simulink model "LEDblink_v02"  (Simulink 7.1)
settings: Solver=FixedStepDiscrete  StartTime=0.0  StopTime=10.0  FixedStep=0.001  RelTol=1e-3
libraries: dsPICdrivers x4, simulink x1
settings Model: Creator=Lubin  LastModifiedBy=Lubin
settings OptimizationCC: OptimizeModelRefInitCode=on  LifeSpan=1
settings DebuggingCC: SaveWithParameterizedLinksMsg=none  SignalResolutionControl=TryResolveAllWithWarning  MultiTaskDSMMsg=warning  MultiTaskCondExecSysMsg=none
settings HardwareCC: ProdBitPerInt=16  ProdEndianess=LittleEndian  ProdWordSize=16  ProdHWDeviceType=16-bit Generic
settings RTWCC: SystemTargetFile=dspic.tlc  TemplateMakefile=dspic_pic30_gcc.tmf  Description=Embedded Target for Microchip dsPIC (real-time)  ProcessScript=dspic_make_rtw_hook  IncludeERTFirstTime=on
settings CodeAppCC: IgnoreCustomStorageClasses=off
settings STFCustomTargetCC: TargetFcnLib=ansi_tfl_tmw.mat  ModelReferenceCompliant=off  IncludeMdlTerminateFcn=off  CombineOutputUpdateFcns=on  SuppressErrorStatus=on  ERTCustomFileBanners=on  SupportContinuousTime=off  SupportNonInlinedSFcns=off  SystemTargetFile=dspic.tlc
settings ERTTargetCC: TargetFcnLib=ansi_tfl_tmw.mat  ModelReferenceCompliant=off  CompOptLevelCompliant=off  IncludeMdlTerminateFcn=off  SuppressErrorStatus=on  ERTFirstTimeCompliant=off  ModelStepFunctionPrototypeControlCompliant=off  InlinedParameterPlacement=NonHierarchical  ERTSrcFileBannerTemplate=dsPIC_code_template.cgt  ERTHdrFileBannerTemplate=dsPIC_code_template.cgt  ERTDataSrcFileTemplate=dsPIC_code_template.cgt  ERTDataHdrFileTemplate=dsPIC_code_template.cgt  ERTCustomFileTemplate=dsPIC_main.tlc
settings CustomProperty: DataType=string  Value=C:\PROGRA~1\MATLAB71\rtw\bin\win32\gmake

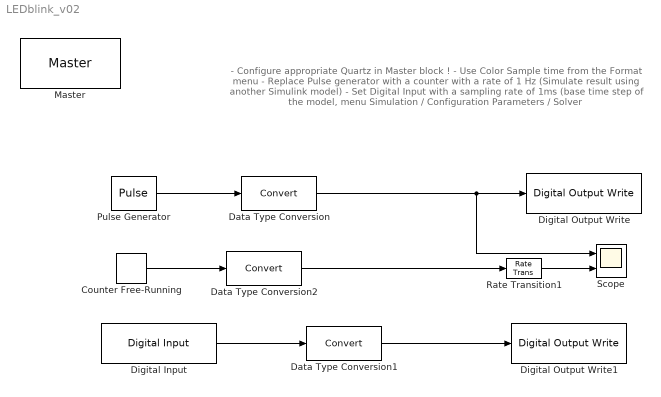
== system LEDblink_v02 ==
  note: - Configure appropriate Quartz in Master block !
      | - Use Color Sample time from the Format menu
      | - Replace Pulse generator with a counter with a rate of 1 Hz (Simulate result using another Simulink model)
      | - Set Digital Input with a sampling rate of 1ms (base time step of the model, menu  Simulation / Configuration Parameters / Solver
  Counter Free-Running : simulink/Sources/Counter Free-Running  SystemSampleTime=-1  NumBits=1  tsamp=1
  Data Type Conversion : DataTypeConversion  OutDataType=sfix(16)  OutScaling=2^0
  Data Type Conversion1 : DataTypeConversion  OutDataType=sfix(16)  OutScaling=2^0
  Data Type Conversion2 : DataTypeConversion  OutDataType=sfix(16)  OutScaling=2^0
  Digital Input : dsPICdrivers/Digital I//O/Digital Input  Tag=dsPIC_Digital_Input  PORT=B  Pin=[1]  SampleTime=.001  OrderingInOutPopup=None
  Digital Output Write : dsPICdrivers/Digital I//O/Digital Output Write  Tag=dsPIC_Digital_Output  Priority=5  PORT=F  Pin=[2]  Simultaneous=off  OrderingInOutPopup=None
  Digital Output Write1 : dsPICdrivers/Digital I//O/Digital Output Write  Tag=dsPIC_Digital_Output  Priority=5  PORT=D  Pin=[2]  Simultaneous=on  OrderingInOutPopup=None
  Master : dsPICdrivers/Master  Tag=dsPIC_MASTER  Priority=1  TimeStepType=Timer1  picType=24fJ64GA006  fcy=2500000  Quartz_33f=5e6  PLLActive_33f=off  fcyDesired_33f=0  tmr1="[1  2499  0]"  tmr1Info="Time Step : 0.001  ;   Error : 0%  PR1=2499"  tmr2345="[0  0  0  0]"  tmr2345cfg=[-1 -1 -1 -1]  IOautoConf=on  typePort="[ 0   0   0   0   0   0   0   0   0   0   0   0   0   0   0   0   0   9   0   0   0   0   0   0   0   0   0   0   0   0   0   0   0   0   0   0   0   0   0   0   0   0   0   0   0   0   0   0   0   0  10   0   0   0   0   0   0   0   0   0   0   0   0   0   0   0   0   0   0   0   0   0   0   0   0   0   0   0   0   0   0   0  10   0   0   0   0   0   0   0   0   0   0   0   0   0   0   0   0   0   0   0   0   0   0   0   0   0   0   0   0   0 ]"  TRIS="[ 65535  65535  65535  65531  65535  65531  65535 ]"  ADPCFG=2  MasterBusyPort=None  MasterOverloadPort=None  FOSC=Quartz (XT - HS)  TempProtection_33f=TEMP_ON  FPBOR=<empty>  PWRT=disable  MCLR=<empty>  PowerSave=off
  Pulse Generator : DiscretePulseGenerator  Period=100  PulseWidth=50  SampleTime=0.01
  Rate Transition1 : RateTransition
  Scope : Scope  NumInputPorts=2
      settings: YMin=-5~-5  YMax=5~5
  wires:
  Data Type Conversion/1 -> Digital Output Write/1, Scope/1
  Digital Input/1 -> Data Type Conversion1/1
  Data Type Conversion1/1 -> Digital Output Write1/1
  Pulse Generator/1 -> Data Type Conversion/1
  Counter Free-Running/1 -> Data Type Conversion2/1
  Data Type Conversion2/1 -> Rate Transition1/1
  Rate Transition1/1 -> Scope/2
